simulink model "integral_lqr_tracking"  (R2025b)
settings: Solver=ode45  StartTime=0.0  StopTime=t_sim  MaxStep=1e-3*Ts  MinStep=1e-4*Ts  RelTol=1e-3
undefined symbols (not defined in the file): C, DiscIntNeverNeededParam, K_q, K_x, Ts, x0i
libraries: cstblocks x1
settings Model: Creator=davidecovolo  LastModifiedBy=ABBAS MANSOUR
settings SolverCC: InitialStep=1e-4*Ts

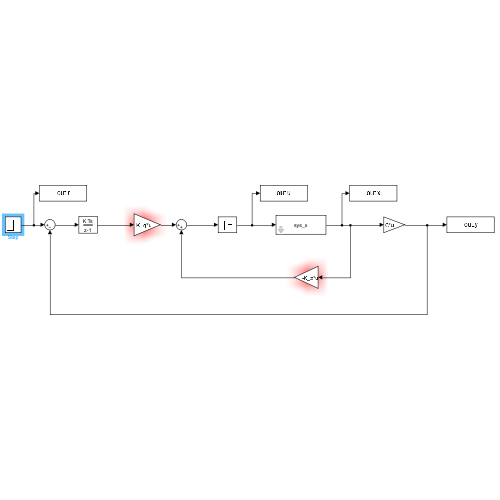
[thumbnail: Simulink's stored preview of the top-level diagram]
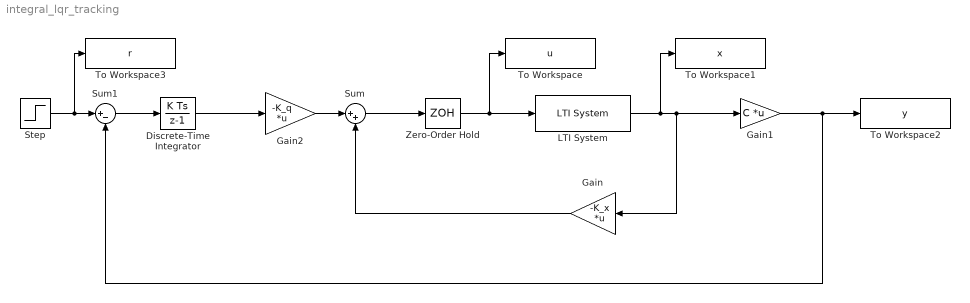
== system integral_lqr_tracking ==
  Discrete-Time Integrator : DiscreteIntegrator  InitialCondition=x0i  SampleTime=Ts  ICPrevOutput=DiscIntNeverNeededParam  ICPrevScaledInput=DiscIntNeverNeededParam
  Gain : Gain  Gain=-K_x  Multiplication=Matrix(K*u)
  Gain1 : Gain  Gain=C  Multiplication=Matrix(K*u)
  Gain2 : Gain  Gain=-K_q  Multiplication=Matrix(K*u)
  LTI System : cstblocks/LTI System  sys=sys_x  IC=x0  PadeOrder=0
  Step : Step  Time=0  SampleTime=Ts
  Sum : Sum  Inputs=|++
  Sum1 : Sum  Inputs=|+-
  To Workspace : ToWorkspace  VariableName=u  SaveFormat=Timeseries  SampleTime=Ts
  To Workspace1 : ToWorkspace  VariableName=x  SaveFormat=Timeseries  SampleTime=Ts
  To Workspace2 : ToWorkspace  VariableName=y  SaveFormat=Timeseries  SampleTime=-1
  To Workspace3 : ToWorkspace  VariableName=r  SaveFormat=Timeseries  SampleTime=Ts
  Zero-Order Hold : ZeroOrderHold  SampleTime=Ts
  wires:
  Gain/1 -> Sum/2
  LTI System/1 -> To Workspace1/1, Gain/1, Gain1/1
  Zero-Order Hold/1 -> To Workspace/1, LTI System/1
  Gain1/1 -> Sum1/2, To Workspace2/1
  Sum/1 -> Zero-Order Hold/1
  Discrete-Time Integrator/1 -> Gain2/1
  Gain2/1 -> Sum/1
  Sum1/1 -> Discrete-Time Integrator/1
  Step/1 -> To Workspace3/1, Sum1/1
